simulink model "pi_speed_control_transfer_function"  (R2024b)
settings: Solver=VariableStepAuto  StartTime=0.0  StopTime=0.4  RelTol=1e-3
undefined symbols (not defined in the file): B_m, J_m, kfi, L_a, R_a, T_nl
settings Model: Creator=kisca  LastModifiedBy=DE MK HU
settings DebuggingCC: UnderspecifiedInitializationDetection=Classic  MergeDetectMultiDrivingBlocksExec=none
settings ModelReferenceCC: PropagateSignalLabelsOutOfModel=off

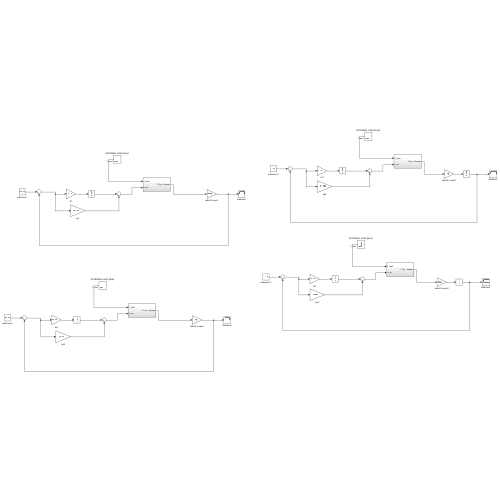
[thumbnail: Simulink's stored preview of the top-level diagram]
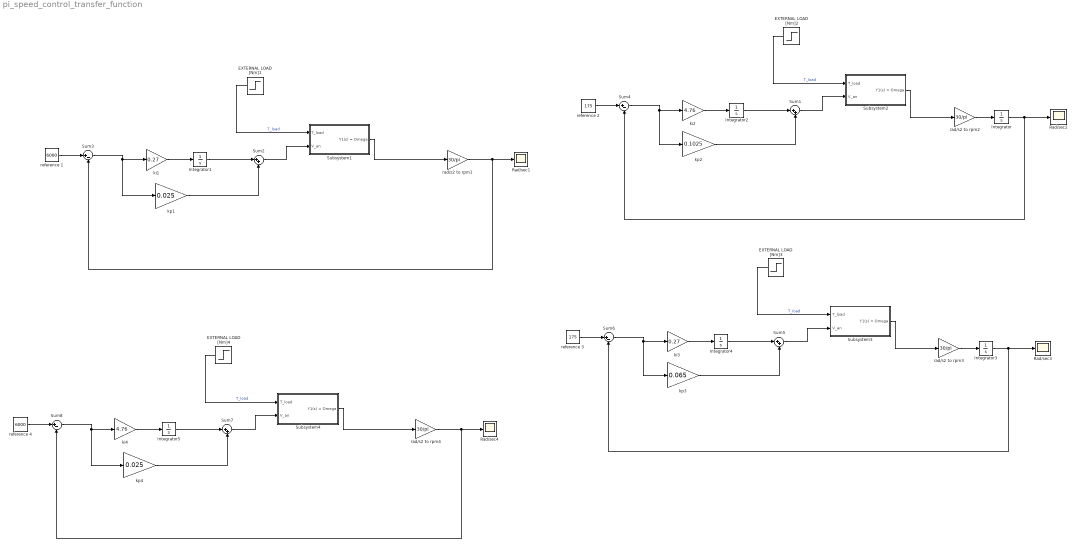
== system pi_speed_control_transfer_function ==
  EXTERNAL LOAD [Nm]{1..4} (4 alike) : Step  Time=0.25  After=T_nl  SampleTime=0
  Integrator{,1..5} (6 alike) : Integrator
  Rad/sec{1..4} (4 alike) : Scope
  Subsystem1 : Subsystem
  Subsystem2 : Subsystem
  Subsystem3 : Subsystem
  Subsystem4 : Subsystem
  Sum{1..2,5,7} (4 alike) : Sum  Inputs=|++
  Sum{3..4,6,8} (4 alike) : Sum  Inputs=|+-
  ki1 : Gain  Gain=0.27
  ki2 : Gain  Gain=4.76
  ki3 : Gain  Gain=0.27
  ki4 : Gain  Gain=4.76
  kp1 : Gain  Gain=0.025
  kp2 : Gain  Gain=0.1025
  kp3 : Gain  Gain=0.065
  kp4 : Gain  Gain=0.025
  rad/s2 to rpm{1..4} (4 alike) : Gain  Gain=30/pi
  reference 1 : Constant  Value=6000
  reference 2 : Constant  Value=175
  reference 3 : Constant  Value=175
  reference 4 : Constant  Value=6000
  wires:
  reference 1/1 -> Sum3/1
  ki1/1 -> Integrator1/1
  Sum2/1 -> Subsystem1/2(V_an)
  Integrator1/1 -> Sum2/1
  kp1/1 -> Sum2/2
  rad/s2 to rpm1/1 -> Sum3/2, Rad/sec1/1
  Sum3/1 -> kp1/1, ki1/1
  EXTERNAL LOAD [Nm]1/1 -> Subsystem1/1(T_load)  "T_load"
  Subsystem1/1(Y1(s) = Omega) -> rad/s2 to rpm1/1
  Integrator2/1 -> Sum1/1
  reference 2/1 -> Sum4/1
  Sum1/1 -> Subsystem2/2(V_an)
  ki2/1 -> Integrator2/1
  EXTERNAL LOAD [Nm]2/1 -> Subsystem2/1(T_load)  "T_load"
  Subsystem2/1(Y1(s) = Omega) -> rad/s2 to rpm2/1
  Sum4/1 -> kp2/1, ki2/1
  kp2/1 -> Sum1/2
  rad/s2 to rpm2/1 -> Integrator/1
  Integrator/1 -> Rad/sec2/1, Sum4/2
  rad/s2 to rpm3/1 -> Integrator3/1
  Sum6/1 -> kp3/1, ki3/1
  Integrator3/1 -> Rad/sec3/1, Sum6/2
  reference 3/1 -> Sum6/1
  Integrator4/1 -> Sum5/1
  Subsystem3/1(Y1(s) = Omega) -> rad/s2 to rpm3/1
  ki3/1 -> Integrator4/1
  kp3/1 -> Sum5/2
  Sum5/1 -> Subsystem3/2(V_an)
  EXTERNAL LOAD [Nm]3/1 -> Subsystem3/1(T_load)  "T_load"
  Integrator5/1 -> Sum7/1
  reference 4/1 -> Sum8/1
  Sum7/1 -> Subsystem4/2(V_an)
  ki4/1 -> Integrator5/1
  EXTERNAL LOAD [Nm]4/1 -> Subsystem4/1(T_load)  "T_load"
  Subsystem4/1(Y1(s) = Omega) -> rad/s2 to rpm4/1
  Sum8/1 -> kp4/1, ki4/1
  kp4/1 -> Sum7/2
  rad/s2 to rpm4/1 -> Sum8/2, Rad/sec4/1

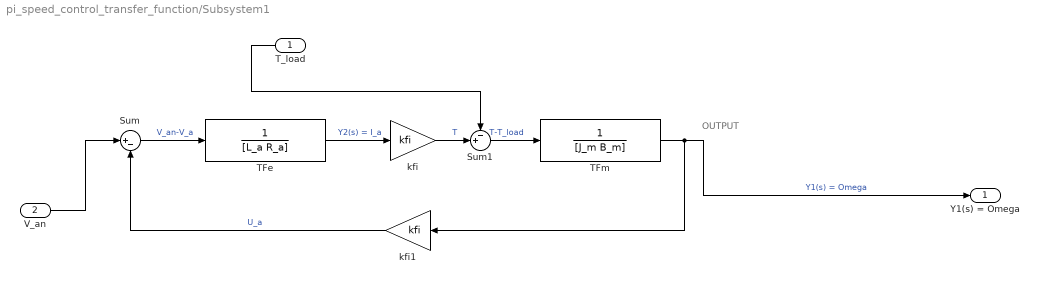
== system pi_speed_control_transfer_function/Subsystem1 ==
  note: OUTPUT
  T_load : Inport
  V_an : Inport  Port=2
  Sum : Sum  Inputs=|+-
  Sum1 : Sum  Inputs=-+|
  TFe : TransferFcn  Denominator=[L_a R_a]
  TFm : TransferFcn  Denominator=[J_m B_m]
  kfi : Gain  Gain=kfi
  kfi1 : Gain  Gain=kfi
  Y1(s) = Omega : Outport
  wires:
  T_load/1 -> Sum1/1
  V_an/1 -> Sum/1
  kfi1/1 -> Sum/2  "U_a"
  TFe/1 -> kfi/1  "Y2(s) = I_a"
  TFm/1 -> Y1(s) = Omega/1, kfi1/1  "Y1(s) = Omega"
  kfi/1 -> Sum1/2  "T"
  Sum/1 -> TFe/1  "V_an-V_a"
  Sum1/1 -> TFm/1  "T-T_load"

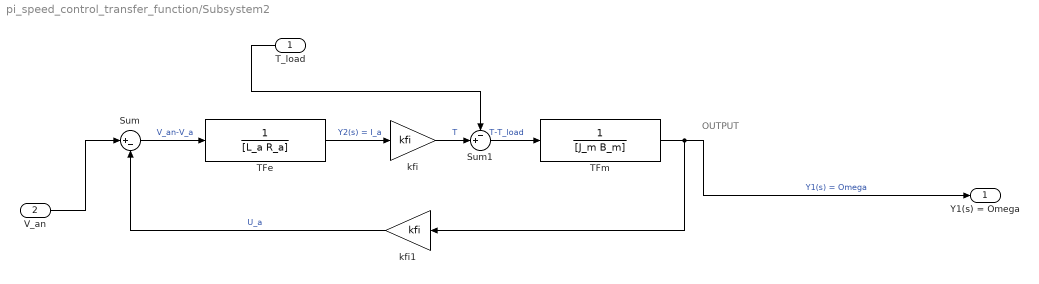
== system pi_speed_control_transfer_function/Subsystem2 ==
  note: OUTPUT
  T_load : Inport
  V_an : Inport  Port=2
  Sum : Sum  Inputs=|+-
  Sum1 : Sum  Inputs=-+|
  TFe : TransferFcn  Denominator=[L_a R_a]
  TFm : TransferFcn  Denominator=[J_m B_m]
  kfi : Gain  Gain=kfi
  kfi1 : Gain  Gain=kfi
  Y1(s) = Omega : Outport
  wires:
  T_load/1 -> Sum1/1
  V_an/1 -> Sum/1
  kfi1/1 -> Sum/2  "U_a"
  TFe/1 -> kfi/1  "Y2(s) = I_a"
  TFm/1 -> Y1(s) = Omega/1, kfi1/1  "Y1(s) = Omega"
  kfi/1 -> Sum1/2  "T"
  Sum/1 -> TFe/1  "V_an-V_a"
  Sum1/1 -> TFm/1  "T-T_load"

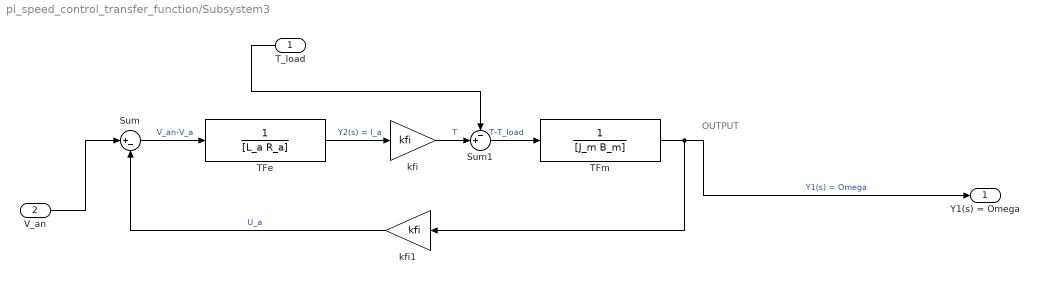
== system pi_speed_control_transfer_function/Subsystem3 ==
  note: OUTPUT
  T_load : Inport
  V_an : Inport  Port=2
  Sum : Sum  Inputs=|+-
  Sum1 : Sum  Inputs=-+|
  TFe : TransferFcn  Denominator=[L_a R_a]
  TFm : TransferFcn  Denominator=[J_m B_m]
  kfi : Gain  Gain=kfi
  kfi1 : Gain  Gain=kfi
  Y1(s) = Omega : Outport
  wires:
  T_load/1 -> Sum1/1
  V_an/1 -> Sum/1
  kfi1/1 -> Sum/2  "U_a"
  TFe/1 -> kfi/1  "Y2(s) = I_a"
  TFm/1 -> Y1(s) = Omega/1, kfi1/1  "Y1(s) = Omega"
  kfi/1 -> Sum1/2  "T"
  Sum/1 -> TFe/1  "V_an-V_a"
  Sum1/1 -> TFm/1  "T-T_load"

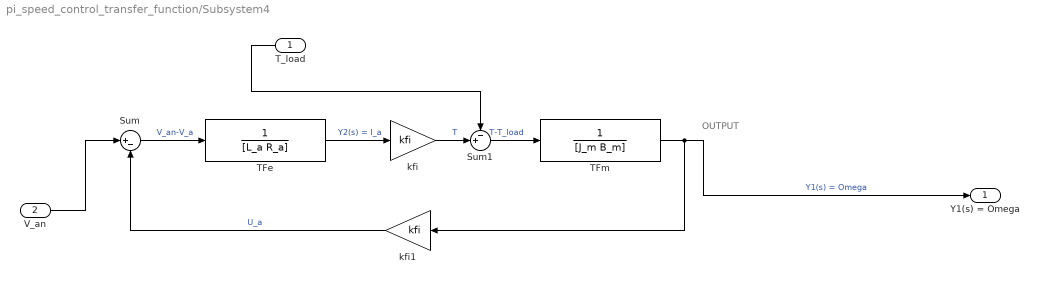
== system pi_speed_control_transfer_function/Subsystem4 ==
  note: OUTPUT
  T_load : Inport
  V_an : Inport  Port=2
  Sum : Sum  Inputs=|+-
  Sum1 : Sum  Inputs=-+|
  TFe : TransferFcn  Denominator=[L_a R_a]
  TFm : TransferFcn  Denominator=[J_m B_m]
  kfi : Gain  Gain=kfi
  kfi1 : Gain  Gain=kfi
  Y1(s) = Omega : Outport
  wires:
  T_load/1 -> Sum1/1
  V_an/1 -> Sum/1
  kfi1/1 -> Sum/2  "U_a"
  TFe/1 -> kfi/1  "Y2(s) = I_a"
  TFm/1 -> Y1(s) = Omega/1, kfi1/1  "Y1(s) = Omega"
  kfi/1 -> Sum1/2  "T"
  Sum/1 -> TFe/1  "V_an-V_a"
  Sum1/1 -> TFm/1  "T-T_load"
